simulink model "turbo_controller"  (R2025a)
settings: Solver=FixedStepAuto  StartTime=0.0  StopTime=inf  FixedStep=0.001  RelTol=1e-3
PostLoadFcn:
  | % 自动定位同目录CubeMX文件；不需要外部初始化脚本。
  | codertarget.data.setParameterValue('turbo_controller','STM32CubeMX.ProjectFile',fullfile(fileparts(get_param('turbo_controller','FileName')),'turbo_f407.ioc'));
InitFcn:
  | % 中文说明：按原控制器字段与类型创建三组接口总线；控制参数已内嵌。
  | tc_names=["EValve_Cycle" "EValve_Open" "Eblast_Cycle" "Eblast_Open" "Motor_Cycle" "Motor_Open" "EValve_Enable" "Eblast_Enable" "Motor_Enable" "SWO_Firework" "SWO_BleedAir" "EngineState" "Flag_ECUReset_Clear" "Flag_ECUReset_Save" "Flag_Reset_Enable" "Accelerator" "Nc_dem" "Nc"]; tc_types=["uint16" "uint16" "uint16" "uint16" "uint16" "uint16" "uint8" "uint8" "uint8" "uint8" "uint8" "uint8" "uint8" "uint8" "uint8" "single" "single" "single"];
  | for tc_k=1:numel(tc_names)
  |  tc_e(tc_k)=Simulink.BusElement; tc_e(tc_k).Name=char(tc_names(tc_k)); tc_e(tc_k).DataType=char(tc_types(tc_k));
  | end
  | EngineControl_Out=Simulink.Bus; EngineControl_Out.DataScope='Exported'; EngineControl_Out.Elements=tc_e;
  | clear tc_e tc_names tc_types tc_k
  | tc_names=["savedata1" "savedata2" "savedata3" "savedata4" "savedata5" "savedata6" "savedata7" "savedata8" "savedata9" "savedata10" "savedata11" "savedata12" "savedata13" "savedata14" "savedata15" "savedata16" "savedata17" "savedata18" "savedata19" "savedata20" "savedata21" "savedata22" "savedata23" "savedata24" "savedata25"]; tc_types=["single" "single" "single" "single" "single" "single" "single" "single" "single" "single" "single" "single" "single" "single" "single" "single" "single" "single" "single" "single" "single" "single" "single" "single" "single"];
  | for tc_k=1:numel(tc_names)
  |  tc_e(tc_k)=Simulink.BusElement; tc_e(tc_k).Name=char(tc_names(tc_k)); tc_e(tc_k).DataType=char(tc_types(tc_k));
  | end
  | SaveData_Out=Simulink.Bus; SaveData_Out.DataScope='Exported'; SaveData_Out.Elements=tc_e;
  | clear tc_e tc_names tc_types tc_k
  | tc_names=["senddata1" "senddata2" "senddata3" "senddata4" "senddata5" "senddata6" "senddata7" "senddata8" "senddata9" "senddata10" "senddata11" "senddata12" "senddata13" "senddata14" "senddata15" "senddata16" "senddata17" "senddata18" "senddata19" "senddata20" "senddata21" "senddata22" "senddata23" "senddata24" "senddata25" "senddata26" "senddata27" "senddata28" "senddata29"]; tc_types=["uint8" "uint8" "uint8" "uint8" "uint8" "uint8" "uint8" "uint8" "uint8" "uint8" "uint8" "uint8" "uint8" "uint8" "uint8" "uint8" "uint8" "uint8" "uint8" "uint8" "uint8" "uint8" "uint8" "uint8" "uint8" "uint8" "uint8" "uint8" "uint8"];
  | for tc_k=1:numel(tc_names)
  |  tc_e(tc_k)=Simulink.BusElement; tc_e(tc_k).Name=char(tc_names(tc_k)); tc_e(tc_k).DataType=char(tc_types(tc_k));
  | end
  | SendData_Out=Simulink.Bus; SendData_Out.DataScope='Exported'; SendData_Out.Elements=tc_e;
  | clear tc_e tc_names tc_types tc_k
  | 
  | % 以下为接口中文说明；只设置描述，不改变数值或数据类型。
  | EngineControl_Out.Description='执行控制输出（阀、电机、点火、状态及复位请求）';
  | tc_cn=["EValve_Cycle（主油阀周期计数（每计数2毫秒））" "EValve_Open（主油阀开通计数（每计数2毫秒））" "Eblast_Cycle（副油阀周期计数（每计数2毫秒））" "Eblast_Open（副油阀开通计数（每计数2毫秒））" "Motor_Cycle（起动电机周期计数）" "Motor_Open（起动电机开通计数）" "EValve_Enable（主油阀驱动使能）" "Eblast_Enable（副油阀驱动使能）" "Motor_Enable（起动电机使能）" "SWO_Firework（点火器使能（1开））" "SWO_BleedAir（引气阀使能（1开））" "EngineState（发动机状态）" "Flag_ECUReset_Clear（清除复位恢复状态请求）" "Flag_ECUReset_Save（保存复位恢复数据请求）" "Flag_Reset_Enable（处理器软件复位请求）" "Accelerator（油门／油泵给定控制量）" "Nc_dem（控制目标转速）" "Nc（发动机反馈转速（转每分））"];
  | tc_elements=EngineControl_Out.Elements;
  | for tc_k=1:numel(tc_cn)
  |  tc_elements(tc_k).Description=char(tc_cn(tc_k));
  | end
  | EngineControl_Out.Elements=tc_elements;
  | clear tc_cn tc_elements tc_k
  | SaveData_Out.Description='25项运行记录；字段含义按当前模型数据来源解释';
  | tc_cn=["savedata1（指令回显记录）" "savedata2（入口总温记录（℃））" "savedata3（电源电压记录）" "savedata4（排气温度记录（℃））" "savedata5（标定燃油压力记录）" "savedata6（副油阀占空比记录（％））" "savedata7（主油阀占空比记录（％））" "savedata8（温度修正转速记录）" "savedata9（开关输出及反馈位域）" "savedata10（物理转速记录）" "savedata11（油泵目标给定原始值）" "savedata12（起动电机占空比记录（％））" "savedata13（发动机状态码记录）" "savedata14（故障告警位域记录）" "savedata15（模型记录帧序号）" "savedata16（处理器温度记录（℃））" "savedata17（装订转速记录（沿用旧电源字段名））" "savedata18（导航高度记录）" "savedata19（飞行空速记录）" "savedata20（主阀旧记录位（恒零保留））" "savedata21（第21项保留记录（恒零））" "savedata22（保留记录项22）" "savedata23（保留记录项23）" "savedata24（保留记录项24）" "savedata25（保留记录项25）"];
  | tc_elements=SaveData_Out.Elements;
  | for tc_k=1:numel(tc_cn)
  |  tc_elements(tc_k).Description=char(tc_cn(tc_k));
  | end
  | SaveData_Out.Elements=tc_elements;
  | clear tc_cn tc_elements tc_k
  | SendData_Out.Description='29字段回传及外设命令接口；板端上位机帧只取第3至27字段';
  | tc_cn=["senddata1（回传发送允许标志（不直接上线路））" "senddata2（回传载荷长度25字节）" "senddata3（回传指令回显字节）" "senddata4（总温编码字节（℃＋80））" "senddata5（电源电压编码字节）" "senddata6（排温编码高字节）" "senddata7（排温编码低字节）" "senddata8（燃油压力编码高字节）" "senddata9（燃油压力编码低字节）" "senddata10（副油阀占空比字节（％））" "senddata11（主油阀占空比字节（％））" "senddata12（修正转速编码高字节）" "senddata13（修正转速编码低字节）" "senddata14（驱动及反馈状态位域）" "senddata15（物理转速编码高字节）" "senddata16（物理转速编码低字节）" "senddata17（油泵目标给定高字节（串口二使用））" "senddata18（油泵目标给定低字节（串口二使用））" "senddata19（起动电机占空比命令（串口一使用））" "senddata20（发动机状态码字节）" "senddata21（故障告警位域字节）" "senddata22（帧序号占位（板端另行填写））" "senddata23（处理器温度编码（℃＋50））" "senddata24（控制目标转速编码高字节）" "senddata25（控制目标转速编码低字节）" "senddata26（占位字节（板端改填实测泵速高字节））" "senddata27（占位字节（板端改填实测泵速低字节））" "senddata28（装订转速高字节（本板未发送））" "senddata29（装订转速低字节（本板未发送））"];
  | tc_elements=SendData_Out.Elements;
  | for tc_k=1:numel(tc_cn)
  |  tc_elements(tc_k).Description=char(tc_cn(tc_k));
  | end
  | SendData_Out.Elements=tc_elements;
  | clear tc_cn tc_elements tc_k
  | 
  | 
  | % FRAM模块化事务：接口类型和上电初始状态，随模型保存，无外部初始化文件。
  | clear FM_elements
  | FM_elements(1)=Simulink.BusElement;FM_elements(1).Name='phase';FM_elements(1).DataType='uint8';FM_elements(1).Dimensions=[1 1];FM_elements(1).Description='phase（当前事务阶段）';
  | FM_elements(2)=Simulink.BusElement;FM_elements(2).Name='a';FM_elements(2).DataType='uint8';FM_elements(2).Dimensions=[64 1];FM_elements(2).Description='a（启动时缓存的首区64字节）';
  | FM_elements(3)=Simulink.BusElement;FM_elements(3).Name='active';FM_elements(3).DataType='uint16';FM_elements(3).Dimensions=[1 1];FM_elements(3).Description='active（当前有效记录区地址）';
  | FM_elements(4)=Simulink.BusElement;FM_elements(4).Name='generation';FM_elements(4).DataType='uint32';FM_elements(4).Dimensions=[1 1];FM_elements(4).Description='generation（当前有效记录代号）';
  | FM_elements(5)=Simulink.BusElement;FM_elements(5).Name='record';FM_elements(5).DataType='uint8';FM_elements(5).Dimensions=[64 1];FM_elements(5).Description='record（本次冻结的待写记录）';
  | FM_elements(6)=Simulink.BusElement;FM_elements(6).Name='addr';FM_elements(6).DataType='uint16';FM_elements(6).Dimensions=[1 1];FM_elements(6).Description='addr（本次备用写入地址）';
  | FM_elements(7)=Simulink.BusElement;FM_elements(7).Name='lastSave';FM_elements(7).DataType='single';FM_elements(7).Dimensions=[1 1];FM_elements(7).Description='lastSave（上次开始保存的秒数）';
  | FM_elements(8)=Simulink.BusElement;FM_elements(8).Name='lastState';FM_elements(8).DataType='uint8';FM_elements(8).Dimensions=[1 1];FM_elements(8).Description='lastState（上次保存时的发动机状态）';
  | FM_elements(9)=Simulink.BusElement;FM_elements(9).Name='boot';FM_elements(9).DataType='boolean';FM_elements(9).Dimensions=[1 1];FM_elements(9).Description='boot（启动记录是否允许恢复）';
  | FM_elements(10)=Simulink.BusElement;FM_elements(10).Name='consumed';FM_elements(10).DataType='boolean';FM_elements(10).Dimensions=[1 1];FM_elements(10).Description='consumed（本次启动恢复通知是否已发送）';
  | FM_elements(11)=Simulink.BusElement;FM_elements(11).Name='payload';FM_elements(11).DataType='uint8';FM_elements(11).Dimensions=[20 1];FM_elements(11).Description='payload（当前20字节恢复内容）';
  | ... (+35 lines)
model workspace (MAT data in the model file):
  CRC16_Table_Reference = [0 4129 8258 12387 16516 20645 24774 28903 33032 37161 41290 45419 ... (256 elements, 256x1)]
  PE_Kaer = [0.15402 0.15402 0.12264 0.10076 0.09481 0.07601 0.07111 0.0569 0.05198 0.04926 0.05308 0.04325 ... (13 elements, 1x13)]
  PE_Nr = [21.2982 61.4260372 67.7475458 72.7394382 76.845934 80.6988798 83.8449282 86.6491912 88.9382406 89.178606 91.1938214 93.4068058 ... (13 elements, 1x13)]
  PE_Pump_Translate = 33.5999984741
  PE_RotaSpeed_Translate = 860
  PE_Taer = [0.4939154 0.4939154 0.40780982 0.34066978 0.31622756 0.30405716 0.34300244 0.26785022 0.37393554 0.23914836 0.44563948 0.31044662 ... (13 elements, 1x13)]
  PF_ACCFULLRANGE = 3360
  PF_Flag_ECUReset = 0
  PF_Flag_rx_suc = 1
  PF_Gear_Info = [40000; 45000; 50000; 55000; 57000; 59000; 60000; 61000; 61000; 61000; 61000; 61000]
  PF_K_TiaoJie = 1
  PF_Kpu = 10
  PF_MySet_Rxdata = [0 0 0 0 0 0 0 0 0 0 0 0 ... (50 elements, 50x1)]
  PF_MyUsart1_Rxdata = [0 0 0 0 0 0 0 0 0 0 0 0 ... (50 elements, 50x1)]
  PF_MyUsart2_Rxdata = [0 0 0 0 0 0 0 0 0 0 0 0 ... (50 elements, 50x1)]
  PF_Reset_Information = [0 0 0 0 0 0 0 0 0 0 0 0 ... (20 elements, 20x1)]
  PF_Sensor_X1_T4 = [0 4095]
  PF_Sensor_X2_T4 = [0 1.66666698456]
  PF_Sensor_X3_T4 = [0 504 999 1497 2010 2529 3051 3568 4076 4571 4959]
  PF_Sensor_X_P2 = [0.5 3]
  PF_Sensor_X_Poil = [0.5 3]
  PF_Sensor_X_T1t = [-50 300]
  PF_Sensor_X_Vpower = [0 3]
  PF_Sensor_X_Vpump = [0 3]
  PF_Sensor_Y1_T4 = [0 3]
  PF_Sensor_Y2_T4 = [0 5000]
  PF_Sensor_Y3_T4 = [0 100 200 300 400 500 600 700 800 900 980]
  PF_Sensor_Y_P2 = [0 1000]
  PF_Sensor_Y_Poil = [0 1000]
  PF_Sensor_Y_T1t = [-50 300]
  PF_Sensor_Y_Vpower = [0 33]
  PF_Sensor_Y_Vpump = [0 33]
  PG_CtrlMode_CloseLoop : mpt.Parameter (value not decoded)
  PG_CtrlMode_ManualAcc : mpt.Parameter (value not decoded)
  PG_CtrlMode_Origin : mpt.Parameter (value not decoded)
  PG_CtrlMode_Start : mpt.Parameter (value not decoded)
  PG_CtrlMode_Stop : mpt.Parameter (value not decoded)
  PG_ES_Clp : mpt.Parameter (value not decoded)
  PG_ES_EngStart : mpt.Parameter (value not decoded)
  PG_ES_Manual : mpt.Parameter (value not decoded)
  PG_ES_Origin : mpt.Parameter (value not decoded)
  PG_ES_Stop : mpt.Parameter (value not decoded)
  PG_Instr_BleedAirSet : mpt.Parameter (value not decoded)
  PG_Instr_CloseLoop : mpt.Parameter (value not decoded)
  PG_Instr_ECUReSet : mpt.Parameter (value not decoded)
  PG_Instr_EValveSet : mpt.Parameter (value not decoded)
  PG_Instr_EblastSet : mpt.Parameter (value not decoded)
  PG_Instr_Erase : mpt.Parameter (value not decoded)
  PG_Instr_FireWorkSet : mpt.Parameter (value not decoded)
  PG_Instr_ManualPlus : mpt.Parameter (value not decoded)
  PG_Instr_ManualrReduce : mpt.Parameter (value not decoded)
  PG_Instr_MotorSet : mpt.Parameter (value not decoded)
  PG_Instr_OilSet : mpt.Parameter (value not decoded)
  PG_Instr_SelfCheck : mpt.Parameter (value not decoded)
  PG_Instr_Start : mpt.Parameter (value not decoded)
  PG_Instr_Stop : mpt.Parameter (value not decoded)
  PG_Instr_StopZero : Simulink.Parameter (value not decoded)
  PG_Location_Air : Simulink.Parameter (value not decoded)
  PG_Location_Gnd : Simulink.Parameter (value not decoded)
  PG_ServoCtrlMode_CloseLoop : Simulink.Parameter (value not decoded)
  PG_ServoCtrlMode_CloseLoopMax : Simulink.Parameter (value not decoded)
  PG_ServoCtrlMode_CloseLoopMin : Simulink.Parameter (value not decoded)
  PG_ServoCtrlMode_ManualAcc : Simulink.Parameter (value not decoded)
  PG_ServoCtrlMode_ManualAccMax : Simulink.Parameter (value not decoded)
  PG_ServoCtrlMode_ManualAccMin : Simulink.Parameter (value not decoded)
  PG_SpeedDot_Permit : Simulink.Parameter (value not decoded)
  PL_EngineModel_Actuator = [0 10 100]
  PL_EngineModel_EngineStar_Press_P2 = [1013 1098.4 1099.144828 1099.931034 1103.613793 1162.662069 1143.793103 1131.006897 1123.186207 1117.6 1114 1111.806897 ... (127 elements, 1x127)]
  PL_EngineModel_EngineStar_RotaSpeed = [200 2000 9584 9660 10220 10240 10260 10288 10308 10368 10380 10408 ... (127 elements, 1x127)]
  PL_EngineModel_EngineStar_Temp_Exhaust = [128 129 129.1 130 131 131.1 132 133 134 134.1 135 135.1 ... (127 elements, 1x127)]
  PL_EngineModel_EngineStar_Time = [0.05 0.1 0.15 0.2 0.25 0.3 0.35 0.4 0.45 0.5 0.55 0.6 ... (127 elements, 1x127)]
  PL_EngineModel_IdleAbove_Nr = [0 21.2982 61.4260372 67.7475458 72.7394382 76.845934 80.6988798 83.8449282 86.6491912 88.9382406 89.178606 91.1938214 ... (14 elements, 1x14)]
  PL_EngineModel_IdleAbove_P2r = [0.986923266716 1.57907722675 1.81593881076 1.99358499877 2.23044658278 2.43770046879 2.65482358747 2.84233900814 3.03972366149 3.18776215149 3.25684678016 3.3950160375 ... (14 elements, 1x14)]
  PL_EngineModel_IdleAbove_Tempr = [0.0536001429337 1.07200285867 1.63301768805 1.63659103091 1.66875111667 1.72592460247 1.77595140254 1.86171163123 1.95461854565 2.03323208862 2.03323208862 2.13685903162 ... (14 elements, 1x14)]
  PL_EngineModel_IdleAbove_Ter = [0.42434128 0.42434128 0.42434128 0.30669408 0.23570008 0.22150128 0.1997974 0.23803274 0.16115638 0.24279948 0.13600422 0.31308354 ... (14 elements, 1x14)]
  PL_EngineModel_IdleAbove_Wfr = [0 10.142 23.8337 27.8905 31.9473 36.0041 40.0609 44.1177 48.1745 52.2313 52.7384 56.7952 ... (14 elements, 1x14)]
  PL_EngineModel_Press_P2 = [400 400 400 400 400 400 400 400 400 400]
  PL_EngineModel_Rotaspeed = [0 20000 96400]
  PL_EngineModel_Temp_Exhaust = [500 500 500 500 500 500 500 500 500 500]
  PL_Kaer = [0.1 0.1 0.1 0.1 0.1 0.1]
  PL_Nr = [50 60 70 80 90 100]
  PL_Taer = [0.1 0.1 0.1 0.1 0.1 0.1]
  Sig : Simulink.Signal (value not decoded)
  Ts_ms : Simulink.Parameter (value not decoded)
  false : Simulink.Parameter (value not decoded)
  true : Simulink.Parameter (value not decoded)
symbols that are objects in the model workspace (value not decoded): PG_CtrlMode_CloseLoop, PG_CtrlMode_ManualAcc, PG_CtrlMode_Origin, PG_CtrlMode_Start, PG_CtrlMode_Stop, PG_ES_Clp, PG_ES_EngStart, PG_ES_Manual, PG_ES_Origin, PG_ES_Stop, PG_Instr_BleedAirSet, PG_Instr_CloseLoop, PG_Instr_EblastSet, PG_Instr_ECUReSet, PG_Instr_Erase, PG_Instr_EValveSet, PG_Instr_FireWorkSet, PG_Instr_ManualPlus, PG_Instr_ManualrReduce, PG_Instr_MotorSet, PG_Instr_OilSet, PG_Instr_SelfCheck, PG_Instr_Start, PG_Instr_Stop, PG_Instr_StopZero, PG_ServoCtrlMode_CloseLoop, PG_ServoCtrlMode_CloseLoopMax, PG_ServoCtrlMode_CloseLoopMin, PG_ServoCtrlMode_ManualAcc, PG_ServoCtrlMode_ManualAccMax, PG_ServoCtrlMode_ManualAccMin, Ts_ms
libraries: simulink x97, stm32blockslib x10, stm32f4xxblockslib x8
(part 10 of 26)

== system turbo_controller/ESM/Flags ==
  note: 把分散的进入条件整理为11个模式转换标志
      |
      | 分别检查初始到起动、初始到手动、进入闭环、各模式停车、停车回初始等条件，再将11个布尔结果打
      | 成Flags总线交状态机使用。
      |
      | 例如普通起动要求Start命令且转速不超过13000；停车回初始要求停车完成且转速不超过20000。部分
      | 控制分支结果先经过一拍延迟再反馈，防止同一拍组合判断互相循环。
      |
      | 这里的每一项是“是否允许这条转换”，不是发动机模式本身，也不是报警编号。真正的当前模式由St
      | ateTranslation保存。
  S_Nc : Inport
      settings: AttributesFormatString=S_Nc（发动机反馈转速（转每分））
  S_Instr : Inport  Port=2
      settings: AttributesFormatString=S_Instr（指令）
  S_Flag_ECUReset : Inport  Port=3
      settings: AttributesFormatString=S_Flag_ECUReset（复位恢复标志）
  S_CLM_Parameter : Inport  Port=4
      settings: AttributesFormatString=S_CLM_Parameter（控制规律管理模块参数）
  Bus Creator1 : BusCreator  Inputs=11
      settings: AttributesFormatString=Bus Creator1（总线创建器1）
  Bus Selector2 : BusSelector  OutputSignals=S_Start（地面起动参数总线）.Flag_RunState（运行状态标志）,S_Stop（停车参数总线）.StopFinish（停车完成标志）
      settings: AttributesFormatString=Bus Selector2（总线选择器2）
  EngineClp : Subsystem  Description=|
      | 产生进入闭环模式的允许条件
      | 
      | 起动分支的阶段结果达到2时，产生Start到Clp条件；手动到Clp使用闭环命令判断；初始到Clp保留复位恢复有效条件。
      | 
      | 同一个“进入闭环”请求，在不同来源模式下有不同条件，不能只看当前目标转速非零就进入闭环。本处只输出转换许可，StateTranslation还要结合当前状态决定采用哪条转换。当前恢复标志上层未启用，恢复进入闭环路径不会自动投入。
      settings: AttributesFormatString=EngineClp（闭环状态转换判定）
  EngineOrigin : Subsystem  Description=|
      | 判断停车结束后是否可以回到初始模式
      | 
      | 只有StopFinish为真，且当前转速Nc≤20000 rpm，两项同时满足才输出Stop2Origin。停车图完成但转速仍很高时，不立即给出这个许可。
      | 
      | 这里不主动制动，也不强迫传感器转速归零。“回初始”是控制流程退出停车模式，不等同于轴已经完全静止。StateTranslation在当前确实处于Stop时才会使用这条转换条件。
      settings: AttributesFormatString=EngineOrigin（原位状态转换判定）
  EngineStart : Subsystem  Description=|
      | 判断能否开始普通起动
      | 
      | 命令必须等于PG_Instr_Start，同时当前转速Nc≤13000 rpm。两项同时成立才输出Origin2Start；其他命令或转速过高时不允许这条转换。
      | 
      | 这只是从初始模式进入普通起动的门槛。点火、建压、供油和退出电机由Start内部顺序图接着执行，不能把13000理解为起动完成转速。工程当前只保留普通Start，不含空气或丙烷起动分支。
      settings: AttributesFormatString=EngineStart（起动状态转换判定）
  EngineStop : Subsystem  Description=|
      | 把停车命令和起动异常转换成停车请求
      | 
      | Stop和StopZero命令都可形成相应停车转换条件；起动内部阶段结果4或15也参与起动转停车判断，用于流程异常或退出。
      | 
      | 分别输出Clp2Stop、Manual2Stop、Start2Stop，交状态机按当前模式选择。内部阶段结果15并不是对外EngineState=15；对外停车模式编号仍为4。
      | 
      | 本模块只提出转换要求，停车后关闭油路、是否短时拖转及何时完成由Stop分支处理。
      settings: AttributesFormatString=EngineStop（停车状态转换判定）
  Manual : Subsystem  Description=|
      | 识别会进入手动模式的八类命令
      | 
      | 比较当前命令是否属于手动泵直接设定、加、减、主油阀、副油阀、起动电机、点火器或引气阀设置。任一匹配便形成进入手动的条件。
      | 
      | 分别向初始、起动、闭环模式提供转Manual标志，真正能用哪一条由状态机的当前状态决定。这里不解释Data6的开度和数值；进入手动后，CLM/Manual才把命令参数换成具体执行器设定。
      settings: AttributesFormatString=Manual（手动）
  Time Delay1 : UnitDelay  SampleTime=-1  HasFrameUpgradeWarning=on
      settings: AttributesFormatString=Time Delay1（时间延迟1）
  Time Delay2 : UnitDelay  SampleTime=-1  HasFrameUpgradeWarning=on
      settings: AttributesFormatString=Time Delay2（时间延迟2）
  Time Delay8 : UnitDelay  SampleTime=-1  HasFrameUpgradeWarning=on
      settings: AttributesFormatString=Time Delay8（时间延迟8）
  S_Flags : Outport
      settings: AttributesFormatString=S_Flags（标志集合）
  wires:
  S_Instr/1 -> EngineStop/2(S_Instr), EngineClp/2(S_Instr), EngineStart/1(S_Instr), Manual/1(S_Instr)
  EngineStart/1(S_Origin2Start) -> [Origin2Start]
  EngineStop/1(S_Clp2Stop) -> [Clp2Stop]
  Manual/1(S_Start2Manual) -> [Start2Manual]
  Manual/2(S_Clp2Manual) -> [Clp2Manual]
  EngineStop/2(S_Manual2Stop) -> [Manual2Stop]
  EngineClp/2(S_Manual2Clp) -> [Manual2Clp]
  S_Flag_ECUReset/1 -> EngineClp/3(S_Flag_ECUReset)
  EngineClp/3(S_Origin2Clp) -> [Origin2Clp]
  EngineStop/3(S_Start2Stop) -> [Start2Stop]
  Manual/3(S_Origin2Manual) -> [Origin2Manual]
  S_CLM_Parameter/1 -> Bus Selector2/1
  Bus Selector2/1 -> Time Delay8/1, Time Delay2/1  "<Flag_RunState（运行状态标志）>"
  Time Delay8/1 -> EngineStop/1(S_Flag_EnigneState)
  EngineClp/1(S_Start2Clp) -> [Start2Clp]
  Time Delay2/1 -> EngineClp/1(S_Flag_EnigneState)
  [Origin2Manual] -> Bus Creator1/11  "Origin2Manual（原位转手动条件）"
  [Origin2Clp] -> Bus Creator1/10  "Origin2Clp（原位转闭环条件）"
  [Start2Stop] -> Bus Creator1/9  "Start2Stop（地面起动转停车条件）"
  [Clp2Manual] -> Bus Creator1/8  "Clp2Manual（闭环转手动条件）"
  [Start2Manual] -> Bus Creator1/7  "Start2Manual（地面起动转手动条件）"
  [Manual2Stop] -> Bus Creator1/6  "Manual2Stop（手动转停车条件）"
  [Manual2Clp] -> Bus Creator1/5  "Manual2Clp（手动转闭环条件）"
  [Stop2Origin] -> Bus Creator1/4  "Stop2Origin（停车转原位条件）"
  [Clp2Stop] -> Bus Creator1/3  "Clp2Stop（闭环转停车条件）"
  [Start2Clp] -> Bus Creator1/2  "Start2Clp（地面起动转闭环条件）"
  [Origin2Start] -> Bus Creator1/1  "Origin2Start（原位转地面起动条件）"
  Bus Selector2/2 -> Time Delay1/1  "<StopFinish（停车完成标志）>"
  Time Delay1/1 -> EngineOrigin/2(S_StopFinish)
  EngineOrigin/1(S_Stop2Origin) -> [Stop2Origin]
  S_Nc/1 -> EngineOrigin/1(S_Nc), EngineStart/2(S_Nc)
  Bus Creator1/1 -> S_Flags/1

== system turbo_controller/ESM/StateTransition ==
  note: 管理发动机运行模式，而不是直接控制驱动电平
      |
      | Flags先根据命令、当前转速、起动阶段结果、停车完成标志及恢复条件，计算允许发生哪些模式转换
      | 。StateTranslation再按当前所在模式和这些允许条件切换状态。
      |
      | 对外只有五种运行模式：Origin=0、Start=1、Clp=2、Manual=3、Stop=4。普通起动内部的A～F及异常
      | 阶段码不属于这五个模式编号。
      |
      | 输出EngineState供CLM选择相应控制分支，供通信与记录解释运行状态。本层不生成泵字节或GPIO脉冲
      | ；转换进入Start仅表示开始执行起动分支，不代表已达到闭环转速。
  S_Flags : Inport
      settings: AttributesFormatString=S_Flags（标志集合）
  Bus Selector1 : BusSelector  OutputSignals=Origin2Start（原位转地面起动条件）,Start2Clp（地面起动转闭环条件）,Clp2Stop（闭环转停车条件）,Stop2Origin（停车转原位条件）,Manual2Clp（手动转闭环条件）,Manual2Stop（手动转停车条件）,Start2Manual（地面起动转手动条件）,Clp2Manual（闭环转手动条件）,Start2Stop（地面起动转停车条件）,Origin2Clp（原位转闭环条件）,Origin2Manual（原位转手动条件）
      settings: AttributesFormatString=Bus Selector1（总线选择器1）
  StateTranslation : Stateflow chart  Description=|  TreatAsAtomicUnit=on
      | 保存五种发动机模式，并按允许条件切换
      | 
      | 初始为Origin，对外编号0。收到相应转换标志后，可以进入普通Start=1、闭环Clp=2或手动Manual=3；运行过程中停车请求进入Stop=4，停车完成并满足转速条件再回Origin。
      | 
      | 每个状态的进入动作写EngineState，其他子系统读取这个编号决定运行哪套控制算法。转换的守卫条件来自Flags，起动是否完成则来自Start内部阶段结果。
      | 
      | 本图是模式记忆：即便某个命令只出现一拍，已进入的模式也会保持到下一次合法转换。不能把命令编号、起动A～F阶段和这五种模式当作同一种“状态”。
      settings: AttributesFormatString=StateTranslation（状态转换）
  S_EngineState : Outport
      settings: AttributesFormatString=S_EngineState（发动机状态）
  wires:
  Bus Selector1/11 -> StateTranslation/11(Origin2Manual)  "<Origin2Manual（原位转手动条件）>"
  Bus Selector1/10 -> StateTranslation/10(Origin2Clp)  "<Origin2Clp（原位转闭环条件）>"
  Bus Selector1/9 -> StateTranslation/9(Start2Stop)  "<Start2Stop（地面起动转停车条件）>"
  Bus Selector1/8 -> StateTranslation/8(Clp2Manual)  "<Clp2Manual（闭环转手动条件）>"
  Bus Selector1/7 -> StateTranslation/7(Start2Manual)  "<Start2Manual（地面起动转手动条件）>"
  Bus Selector1/6 -> StateTranslation/6(Manual2Stop)  "<Manual2Stop（手动转停车条件）>"
  Bus Selector1/5 -> StateTranslation/5(Manual2Clp)  "<Manual2Clp（手动转闭环条件）>"
  StateTranslation/1(EngineState) -> S_EngineState/1
  Bus Selector1/4 -> StateTranslation/4(Stop2Origin)  "<Stop2Origin（停车转原位条件）>"
  Bus Selector1/3 -> StateTranslation/3(Clp2Stop)  "<Clp2Stop（闭环转停车条件）>"
  Bus Selector1/2 -> StateTranslation/2(Start2Clp)  "<Start2Clp（地面起动转闭环条件）>"
  Bus Selector1/1 -> StateTranslation/1(Origin2Start)  "<Origin2Start（原位转地面起动条件）>"
  S_Flags/1 -> Bus Selector1/1

== system turbo_controller/FPM/Subsystem ==
  note: 极值斜率故障
  note: 故障锁存标志
  note: ACDC转速启动前可能乱跳，造成故障锁定
  note: 【本页库子系统中文说明】Detect
      | Change
      | 一、它做什么？
      | 比较当前输入与上一次输入是否不同：发生变化时给出变化标志，不变时不给出变化标
      | 志。它检测的是数值改变，不是判断数值够不够大。内部需要记住上次输入，首次输出
      | 还要结合库块的初值设置。
      | 二、本实例当前参数
      | vinit：0
      | InputProcessing：Elements as channels (sample based)
      | 输出数据类型：布尔值，真或假
      | 三、怎样继续学习？
      | 这是标准库子系统实例。中文说明放在使用它的父级页面，并同步存入本块Descriptio
      | n（模块说明）；官方库链接保留。先看本实例的输入来自哪里、输出交给谁，再结合
      | 以上参数理解作用。
  note: 【本页库子系统中文说明】运行状态
      | 一、它做什么？
      | 这是“过不过这条线”的判断器。将输入与阈值 PG_ES_Clp 作 == 比较，关系成立输
      | 出真（1），否则输出假（0）。例如>=包含恰好等于，>则不包含。它只给出判断标志
      | ，不会自行限幅、报警、切换状态或操作阀门；后续逻辑决定如何使用。名称可能只是
      | 用途提示，实际判据以这里的关系和阈值为准。
      | 二、本实例当前参数
      | 比较关系：==
      | 比较阈值：PG_ES_Clp
      | 输出数据类型：uint8
      | 零交叉检测：开启
      | 三、怎样继续学习？
      | 这是标准库子系统实例。中文说明放在使用它的父级页面，并同步存入本块Descriptio
      | n（模块说明）；官方库链接保留。先看本实例的输入来自哪里、输出交给谁，再结合
      | 以上参数理解作用。
  note: 【本页库子系统中文说明】闭环状态
      | 一、它做什么？
      | 这是“过不过这条线”的判断器。将输入与阈值 PG_ES_Clp 作 == 比较，关系成立输
      | 出真（1），否则输出假（0）。例如>=包含恰好等于，>则不包含。它只给出判断标志
      | ，不会自行限幅、报警、切换状态或操作阀门；后续逻辑决定如何使用。名称可能只是
      | 用途提示，实际判据以这里的关系和阈值为准。
      | 二、本实例当前参数
      | 比较关系：==
      | 比较阈值：PG_ES_Clp
      | 输出数据类型：uint8
      | 零交叉检测：开启
      | 三、怎样继续学习？
      | 这是标准库子系统实例。中文说明放在使用它的父级页面，并同步存入本块Descriptio
      | n（模块说明）；官方库链接保留。先看本实例的输入来自哪里、输出交给谁，再结合
      | 以上参数理解作用。
  note: 区分短时测速异常、持续故障和恢复保存时机
      |
      | 把转速幅值故障与突变故障组合，先形成当前异常，再经10 s定时锁存形成持续故障。暂时异常可让控
      | 制保持，持续异常则允许父级切换备份供油策略。
      |
      | 恢复有效条件持续约2 s后产生恢复工作相关状态；处于闭环时，4 s计时器周期性给出保存事件。模式
      | 变化检测与触发/使能分支产生恢复信息清除请求。
      |
      | 这些都是控制条件，不是FRAM写入已完成的确认。实际保存需要下游事务逐步执行，写失败也不能仅靠
      | 本模块得知。
  note: Detect
      | Change
      | 检测发动机模式是否与上一拍不同
      |
      | 输入为当前模式，与内部保存的上次值比较，变化时输出真，未变化时输出假。初始比较值为0，所以
      | 首次输入0不算变化，首次输入非0会触发。
      |
      | 这是变化事件，不是持续处于某模式的标志。父级用它安排复位恢复信息清除等动作；本实例不直接清
      | 除FRAM，也不会持续一整个模式都重复触发。
  note: 运行状态
      | 运行状态：只判断一个条件
      |
      | 把输入与2比较，使用关系“==”。成立输出1，不成立输出0；输出是判断标志，不是把输入缩放成该
      | 常数。
      |
      | 这里比较的是发动机当前模式：初始0、普通起动1、闭环2、手动3、停车4。结果供父级选择对应控制/
      | 保护路径，不能用命令编号代替模式编号。
  note: 闭环状态
      | 闭环状态：只判断一个条件
      |
      | 把输入与2比较，使用关系“==”。成立输出1，不成立输出0；输出是判断标志，不是把输入缩放成该
      | 常数。
      |
      | 这里比较的是发动机当前模式：初始0、普通起动1、闭环2、手动3、停车4。结果供父级选择对应控制/
      | 保护路径，不能用命令编号代替模式编号。
  In1 : Inport
      settings: AttributesFormatString=In1（输入1）
  In2 : Inport  Port=2
      settings: AttributesFormatString=In2（输入2）
  Bus Selector1 : BusSelector  OutputSignals=Sensor（传感器信息总线）.Nc_Flag_Locking（转速信号锁定标志）,Sensor（传感器信息总线）.Ncdot_Flag_Locking（转速变化率锁定标志）
      settings: AttributesFormatString=Bus Selector1（总线选择器1）
  Bus Selector2 : BusSelector  OutputSignals=COMM（通信信息总线）.Flag_ECUReset_Use（复位恢复数据使用标志）
      settings: AttributesFormatString=Bus Selector2（总线选择器2）
  Constant4 : Constant  Value=10000  OutDataTypeStr=single  SampleTime=-1
      settings: AttributesFormatString=Constant4（常量4）
  Data Type Conversion{1..5} (5 alike) : DataTypeConversion  OutDataTypeStr=uint8  SaturateOnIntegerOverflow=off  RndMeth=Floor
      Data Type Conversion1 settings: AttributesFormatString=Data Type Conversion1（数据类型转换1）
      Data Type Conversion2 settings: AttributesFormatString=Data Type Conversion2（数据类型转换2）
      Data Type Conversion3 settings: AttributesFormatString=Data Type Conversion3（数据类型转换3）
      Data Type Conversion4 settings: AttributesFormatString=Data Type Conversion4（数据类型转换4）
      Data Type Conversion5 settings: AttributesFormatString=Data Type Conversion5（数据类型转换5）
  Detect Change : simulink/Logic and Bit Operations/Detect Change  Description=|  vinit=0  OutDataTypeStr=boolean
      | 检测发动机模式是否与上一拍不同
      | 
      | 输入为当前模式，与内部保存的上次值比较，变化时输出真，未变化时输出假。初始比较值为0，所以首次输入0不算变化，首次输入非0会触发。
      | 
      | 这是变化事件，不是持续处于某模式的标志。父级用它安排复位恢复信息清除等动作；本实例不直接清除FRAM，也不会持续一整个模式都重复触发。
      settings: AttributesFormatString=Detect Change（检测变化）
  Flag_ECUReset_Reset : Subsystem  Description=|  TreatAsAtomicUnit=on
      | 在被触发且允许时提出恢复记录清除请求
      | 
      | 这是带触发和使能的动作子系统。只有父级满足执行条件时，内部常量1才输出为清除请求；不是模型每拍都无条件清除FRAM。
      | 
      | 本处不发送SPI、不擦除整片存储器，只生成逻辑标志。父级将它与模式变化等条件组合，再由FRAM事务层决定实际记录处理。
      settings: AttributesFormatString=Flag_ECUReset_Reset（标志控制器复位复位）
  Hold_2000ms : Stateflow chart  Description=|  TreatAsAtomicUnit=on  RTWFcnName=Timmer  RTWFileName=MCM_Timmer
      | 等待恢复条件持续约2 s后才置恢复控制标志
      | 
      | Flag_ECUReset为真时累计次数，为假时立即清计数并令ResetControl为假。计数尚小于Time_ms/Ts_ms时输出假，达到门限后输出真。
      | 
      | 当前Time_ms=2000、Ts_ms=20，对应100次调用。这样一次瞬时有效信号不会立即完成恢复确认。计数有10000封顶，避免持续有效时无限增长；输入撤销后需要重新累计。
      settings: AttributesFormatString=Hold_2000ms（保持2000毫秒）  RTWFcnNameOpts=Use subsystem name  RTWFileNameOpts=User specified
  Hold_4000ms : Stateflow chart  Description=|  TreatAsAtomicUnit=on  RTWFcnName=Timmer  RTWFileName=MCM_Timmer
      | 闭环期间按约4 s间隔提出保存请求
      | 
      | Flag_ClpControl为真时计数，为假时清零且不保存。当计数严格大于Time_ms/Ts_ms时，ECUReset_Save给出真并清计数，随后重新开始下一轮。
      | 
      | 当前Time_ms=4000、Ts_ms=20，比较门限200次，因采用“>”，事件会比恰好200拍多一个调用量级。它是周期性的保存触发，不是持续4 s都在发写命令。真正的多步FRAM写入由事务子系统完成。
      settings: AttributesFormatString=Hold_4000ms（保持4000毫秒）  RTWFcnNameOpts=Use subsystem name  RTWFileNameOpts=User specified
  Logical Operator1 : Logic  Operator=OR  AllPortsSameDT=off  OutDataTypeStr=boolean
      settings: AttributesFormatString=Logical Operator1（逻辑运算1）
  Logical Operator2 : Logic  Operator=OR  AllPortsSameDT=off  OutDataTypeStr=boolean
      settings: AttributesFormatString=Logical Operator2（逻辑运算2）
  Logical Operator3 : Logic  Operator=NOT  AllPortsSameDT=off  OutDataTypeStr=boolean
      settings: AttributesFormatString=Logical Operator3（逻辑运算3）
  Logical Operator4 : Logic  AllPortsSameDT=off  OutDataTypeStr=boolean
      settings: AttributesFormatString=Logical Operator4（逻辑运算4）
  Logical Operator5 : Logic  AllPortsSameDT=off  OutDataTypeStr=boolean
      settings: AttributesFormatString=Logical Operator5（逻辑运算5）
  Scope : Scope
      settings: AttributesFormatString=Scope（示波器）  ActiveDisplayYMinimum=-0.125  ActiveDisplayYMaximum=1.125  DataLoggingVariableName=ScopeData4
  Timmer_ms_Lock : Stateflow chart  Description=|  TreatAsAtomicUnit=on  RTWFcnName=Timmer  RTWFileName=EngineControl_Timmer
      | 持续异常达到时间门限后锁存故障
      | 
      | 输入In为真或内部Flag_Lock已经为真时计数。计数严格大于Time_ms/Ts_ms后，置Out和Flag_Lock为真。锁存之后，即便外部In恢复为假，也继续维持故障状态，直到模型/图初始化。
      | 
      | 父级Time_ms=10000、Ts_ms=20，门限500次调用，采用“>”判断。这样短暂测速异常先走临时保护，持续约10 s才进入长期故障策略。计数有上限，不无限累加。
      settings: AttributesFormatString=Timmer_ms_Lock（计时器毫秒锁存）  RTWSystemCode=Reusable function  RTWFcnNameOpts=Use subsystem name  RTWFileNameOpts=User specified
  dth = T0-288.1 : Constant  Value=4000  OutDataTypeStr=single  SampleTime=-1
      settings: AttributesFormatString=dth = T0-288.1（固定常量4000（旧名称不参与计算））
  dth = T0-288.5 : Constant  Value=2000  OutDataTypeStr=single  SampleTime=-1
      settings: AttributesFormatString=dth = T0-288.5（固定常量2000（旧名称不参与计算））
  运行状态 : simulink/Logic and Bit Operations/Compare To Constant  Description=|  relop===  const=PG_ES_Clp  OutDataTypeStr=uint8
      | 运行状态：只判断一个条件
      | 
      | 把输入与2比较，使用关系“==”。成立输出1，不成立输出0；输出是判断标志，不是把输入缩放成该常数。
      | 
      | 这里比较的是发动机当前模式：初始0、普通起动1、闭环2、手动3、停车4。结果供父级选择对应控制/保护路径，不能用命令编号代替模式编号。
  闭环状态 : simulink/Logic and Bit Operations/Compare To Constant  Description=|  relop===  const=PG_ES_Clp  OutDataTypeStr=uint8
      | 闭环状态：只判断一个条件
      | 
      | 把输入与2比较，使用关系“==”。成立输出1，不成立输出0；输出是判断标志，不是把输入缩放成该常数。
      | 
      | 这里比较的是发动机当前模式：初始0、普通起动1、闭环2、手动3、停车4。结果供父级选择对应控制/保护路径，不能用命令编号代替模式编号。
  Lock_NcFailure : Outport
      settings: AttributesFormatString=Lock_NcFailure（锁存转速故障）
  Flag_NcFailure1 : Outport  Port=2
      settings: AttributesFormatString=Flag_NcFailure1（标志转速故障1）
  Flag_ECUReset_work : Outport  Port=3
      settings: AttributesFormatString=Flag_ECUReset_work（标志控制器复位工作）
  Flag_ECUReset_Clear : Outport  Port=4
      settings: AttributesFormatString=Flag_ECUReset_Clear（清除复位恢复状态请求）
  Flag_ECUReset_Save : Outport  Port=5
      settings: AttributesFormatString=Flag_ECUReset_Save（保存复位恢复数据请求）
  wires:
  Logical Operator2/1 -> Logical Operator5/2, Logical Operator4/2, Scope/1
  Bus Selector2/1 -> Flag_ECUReset_Reset/Enable, Hold_2000ms/1(Flag_ECUReset)  "<Flag_ECUReset_Use（复位恢复数据使用标志）>"
  In1/1 -> Bus Selector1/1, Bus Selector2/1
  Bus Selector1/1 -> Logical Operator2/1  "<Nc_Flag_Locking（转速信号锁定标志）>"
  Bus Selector1/2 -> Logical Operator2/2  "<Ncdot_Flag_Locking（转速变化率锁定标志）>"
  Hold_2000ms/1(ResetControl) -> Flag_ECUReset_Reset/Trigger, Data Type Conversion1/1
  Flag_ECUReset_Reset/1(S_Flag_ECUReset_Clear) -> Logical Operator1/1
  dth = T0-288.5/1 -> Hold_2000ms/2(Time_ms)
  Detect Change/1 -> Logical Operator1/2
  闭环状态/1 -> Hold_4000ms/1(Flag_ClpControl)
  Hold_4000ms/1(ECUReset_Save) -> Data Type Conversion5/1  "Flag_ECUReset_Save（保存复位恢复数据请求）"
  Data Type Conversion2/1 -> Flag_ECUReset_Clear/1  "Flag_ECUReset_Clear（清除复位恢复状态请求）"
  Logical Operator1/1 -> Data Type Conversion2/1
  dth = T0-288.1/1 -> Hold_4000ms/2(Time_ms)
  Data Type Conversion1/1 -> Flag_ECUReset_work/1  "Flag_ECUReset_work（复位恢复运行标志）"
  Timmer_ms_Lock/1(Out) -> Logical Operator3/1, Data Type Conversion3/1
  Constant4/1 -> Timmer_ms_Lock/2(Time_ms)
  In2/1 -> 运行状态/1, 闭环状态/1, Detect Change/1
  运行状态/1 -> Logical Operator4/1
  Logical Operator4/1 -> Timmer_ms_Lock/1(In)
  Data Type Conversion4/1 -> Flag_NcFailure1/1
  Data Type Conversion5/1 -> Flag_ECUReset_Save/1
  Data Type Conversion3/1 -> Lock_NcFailure/1
  Logical Operator3/1 -> Logical Operator5/1
  Logical Operator5/1 -> Data Type Conversion4/1

== system turbo_controller/SDM/LogicSelection3 ==
  note: 根据条件选择两种检测结果
      |
      | C不为0时输出T，C为0时输出F。父级用它在不同运行条件下选择相应检测结果；不把两路标志相加，也
      | 不保存上次值。
      |
      | 本处只处理选择，具体检测阈值在T4_Check及父级比较模块中。当前整个SDM结果最终接到未使用终止
      | 端，因此此选择不会单独触发实际停车或起动。
  C : Inport
      settings: AttributesFormatString=C（条件输入或阶段编号）
  F : Inport  Port=2
      settings: AttributesFormatString=F（假分支输入）
  T : Inport  Port=3
      settings: AttributesFormatString=T（温度、时间或真分支输入）
  Switch : Switch  Criteria=u2 ~= 0  SaturateOnIntegerOverflow=off  InputSameDT=off
      settings: AttributesFormatString=Switch（开关选择）
  Out : Outport
      settings: AttributesFormatString=Out（输出）
  wires:
  F/1 -> Switch/3
  T/1 -> Switch/1
  C/1 -> Switch/2
  Switch/1 -> Out/1

== system turbo_controller/SDM/T4_Check ==
  note: 用排温是否超过100判断升温条件
      |
      | 读取排温并与100比较，输出该比较条件供SDM组合使用。这里采用已送入本模块的温度量，不直接读取
      | ADC计数，也不重新执行传感器标定。
      |
      | 阈值判断仅表示温度位于门限哪一侧，没有持续2 s确认，也不是完整的点火成功识别。当前SDM输出未
      | 继续参与模式控制，不能把本标志视为已经投入的起动保护。
  In1 : Inport
      settings: AttributesFormatString=In1（输入1）
  Constant7 : Constant  Value=100
      settings: AttributesFormatString=Constant7（常量7）
  Data Type Conversion4 : DataTypeConversion  OutDataTypeStr=uint8  SaturateOnIntegerOverflow=off  RndMeth=Floor
      settings: AttributesFormatString=Data Type Conversion4（数据类型转换4）
  Relational Operator5 : RelationalOperator  Operator=>  OutDataTypeStr=boolean  InputSameDT=off
      settings: AttributesFormatString=Relational Operator5（关系比较运算5）
  Out1 : Outport
      settings: AttributesFormatString=Out1（输出1）
  wires:
  Constant7/1 -> Relational Operator5/2
  In1/1 -> Relational Operator5/1
  Relational Operator5/1 -> Data Type Conversion4/1
  Data Type Conversion4/1 -> Out1/1

== system turbo_controller/BoardInput_输入换算与协议解析/In01_Host（上位机命令解析）/Receive（逐字节组帧与保持有效结果）_108 ==
  note: 上位机接收流程：按1→2→3→4阅读，第5步管理通知时机
      |
      | 这页只保留三个输入、两个输出、一个循环块和五个处理步骤。
      | Rx：接收数组；Count：本批新收到多少字节；ControlTick：20 ms更新许可。
      | Command：最近有效的50项命令；Flag：本次是否通知控制任务有新命令。
      |
      | Step01取一项字节，决定本项有效及何时结束循环。
      | Step02识别AA55并拼14字节，未拼完的数据保留到下次。
      | Step03检查收齐事件及累加、异或校验，给出本次接受事件。
      | Step04有效才更新命令，否则保持上一条；14字节后补36个0。
      | Step05记住是否有新命令，等20 ms许可时输出通知。
      |
      | 三种记忆各管一件事：半帧缓存属于Step02；上一条有效命令属于Step04；尚未报告标志属于Step05。
      | 候选帧、有效命令、通知标志不能混为一谈。
      |
      | Loop让这五步在本次调用内逐字节重复，不是五步各等一个采样周期。Step01的下一序号反馈Loop，达
      | 到本批数量或64项就结束。因此一批能处理多字节，也能连续接受多帧。
      |
      | 本次仅拆分层次，保留原来的循环、类型转换、初值、校验与保持逻辑。点开每一步可看具体例子及输
      | 入输出含义。
  Rx（本次接收字节）_11 : Inport  OutDataTypeStr=uint8
  Count（本次有效字节数）_12 : Inport  Port=2  OutDataTypeStr=uint32
  ControlTick（20毫秒更新许可）_13 : Inport  Port=3  OutDataTypeStr=boolean
  Loop（逐项处理循环）_14 : ForIterator  IterationLimit=64  ExternalIncrement=on  IterationVariableDataType=uint32
  Step01_取字节与循环控制 : Subsystem  Description=|
      | 第一步：从本批数据中逐个取字节，决定何时结束循环
      | 
      | Rx是最多64项的接收数组，Count说明其中前几项是本次新收到的字节。Index是外面Loop提供的当前序号，从1开始；它不是已经收到的帧长度。
      | 
      | 1. 当前字节=Rx(Index)。Index≤Count时，本字节有效；否则只执行保持，不把数组尾部的旧值当作新字节。
      | 2. Index≥Count，或者Index=64，任一成立就输出“本批处理结束”。前者表示本批有效字节用完，后者防止超出64项。
      | 3. 尚未结束时输出下一序号Index+1；结束时输出65，让Loop退出。
      | 
      | 例如Count=3，依次处理数组第1、2、3项；到第3项就结束，不再把第4项作为新数据。Count=0时仍会有一次无效项处理，用于保持命令和处理通知，但不会往帧里加入字节。
      | 
      | 本步骤只负责遍历接收数组；它不判断AA55帧头，不校验，不保存命令。Byte和Active送第二步，Last送第五步，NextIndex反馈Loop。
  Step02_拼帧并记住未收完的数据 : Subsystem  Description=|
      | 第二步：识别帧头、拼满14字节，并记住半帧
      | 
      | 输入是一项字节及“本字节有效”标志。内部Collect按AA、55识别帧头，接着按顺序把后续字节放进14项候选缓存，收齐时给出Complete。
      | 
      | Buffer保存尚未验证的候选内容，Position保存下一项要放的位置。每个字节处理后，新的缓存与位置经过类型转换存回记忆，供下一个字节使用；本批结束时也不清掉，因此可跨接收批次续收。
      | 
      | 例：第一次只收到AA、55及其后6字节，第二次又收到剩余6字节，第二次会继续原位置，直到拼满14字节。无效项不会推进收帧。
      | 
      | 输出“候选帧”只是凑齐的内容，尚不能当命令使用；输出“本字节刚好收齐”是一次完成事件。两者送第三步校验，候选内容也送第四步等待是否接受。
      | 
      | 这里的延迟按循环处理的节奏保存记忆，不是在每个字节之间额外等待1 ms。更细的帧头重同步规则仍在Collect内部，原逻辑未改。
  Step03_检查完整性与双校验 : Subsystem  Description=|
      | 第三步：这一帧既要收齐，也要两种校验都通过
      | 
      | Verify只对已收齐的14字节候选帧作有效性检查。对第1～12字节重新计算：
      | 累加校验=这12字节之和 mod 256；
      | 异或校验=第1字节 XOR 第2字节 XOR … XOR 第12字节。
      | 分别与第13、第14字节比较，两项均匹配才通过。
      | 
      | 最终接受事件=“本字节刚好收齐” AND “Verify通过”。即使Verify保留着上一帧的通过状态，没有本次Complete也不会再次接受旧内容。
      | 
      | 例如数据未收满、累加校验不符、异或校验不符，任意一种都会使本次接受事件为假。为真时通知第四步更新命令，并通知第五步记住有新命令待报告。
      | 
      | 本处检查的是通信内容是否符合校验，不判断某条起动命令在当前发动机状态下是否允许执行；命令解释与模式判断在后面的CMMRead、ESM。
  Step04_只保存通过校验的命令 : Subsystem  Description=|
      | 第四步：只用有效帧更新命令，坏帧不能覆盖好命令
      | 
      | 将14字节候选帧后面补36个0，保持原工程50项命令接口：前14项是收到的帧，15～50项为兼容占位。
      | 
      | 本次接受事件为真：选择这组新命令，并存入Latest；
      | 本次接受事件为假：继续输出Latest记住的旧命令。
      | 
      | 例如上一条有效命令是A，本批又来了校验错误的B，输出仍为A；B不会因为已经凑满14字节就覆盖A。首次尚未接受命令时，沿用原有初始值。
      | 
      | 一个接收批次可能连续有多条有效帧，每接受一条就更新一次，批次结束后输出最后一条。这个50项数组是最近有效结果，不是每次通知就自动清空的队列。
      | 
      | 输出交外层Command。是否让控制任务在本拍使用它，由第五步的通知Flag另行表示。
  Step05_等到20毫秒再通知一次 : Subsystem  Description=|
      | 第五步：记住新命令，等20 ms更新时机再通知
      | 
      | Accepted表示本字节刚接受了有效帧，Fresh表示以前收到了有效帧但尚未报告。两者用OR合成NewSeen：只要其中一个为真，就说明有新命令等着通知。
      | 
      | 输出Flag=ControlTick AND NewSeen，再转成原接口数据类型。ControlTick由外层给出，表示当前到了20 ms更新时机；本步骤自己不计时，也不把秒数当输入。
      | 
      | 记忆更新：只有“本批处理结束 AND ControlTick”同时成立，才把待通知标志清零；其余时候继续保存NewSeen。这样循环尚未处理完时不会过早丢掉通知。
      | 
      | 例：第5 ms收到了有效帧，命令先被第四步保存，待通知状态保持；第20 ms更新许可到来时给出Flag，批次处理结束后清除。若这期间没有新帧，第40 ms不会再通知一次。
      | 
      | 同一更新间隔内收到多帧，通知表示“有更新”，第四步给出最近一条，不为每一帧单独排队。Flag是给控制任务的通知，不是向上位机发送的应答。
  Flag（20毫秒新命令通知）_106 : Outport
  Command（最近有效命令）_107 : Outport  Port=2
  wires:
  Step05_等到20毫秒再通知一次/1(新命令通知) -> Flag（20毫秒新命令通知）_106/1  "20毫秒新命令通知"
  Step04_只保存通过校验的命令/1(最近有效命令_50字节) -> Command（最近有效命令）_107/1  "最近有效命令_50项"
  Step01_取字节与循环控制/4(下一循环序号) -> Loop（逐项处理循环）_14/1  "下一序号或退出值65"
  ControlTick（20毫秒更新许可）_13/1 -> Step05_等到20毫秒再通知一次/3(20毫秒更新许可)  "20毫秒更新许可"
  Step01_取字节与循环控制/3(本批处理结束) -> Step05_等到20毫秒再通知一次/2(本批处理结束)  "本批最后一次循环"
  Step03_检查完整性与双校验/1(本字节接受新命令) -> Step04_只保存通过校验的命令/1(本字节接受新命令), Step05_等到20毫秒再通知一次/1(本字节接受新命令)  "本次接受有效帧"
  Step02_拼帧并记住未收完的数据/1(候选14字节帧) -> Step03_检查完整性与双校验/2(候选14字节帧), Step04_只保存通过校验的命令/2(候选14字节帧)  "候选14字节帧"
  Step02_拼帧并记住未收完的数据/2(本字节刚好收齐) -> Step03_检查完整性与双校验/1(本字节刚好收齐)  "刚好收齐一帧"
  Step01_取字节与循环控制/2(本字节有效) -> Step02_拼帧并记住未收完的数据/2(本字节有效)  "本项有效"
  Step01_取字节与循环控制/1(当前字节) -> Step02_拼帧并记住未收完的数据/1(当前字节)  "本项字节"
  Loop（逐项处理循环）_14/1 -> Step01_取字节与循环控制/3(当前循环序号)  "当前字节序号"
  Count（本次有效字节数）_12/1 -> Step01_取字节与循环控制/2(本批有效字节数)  "本批有效字节数"
  Rx（本次接收字节）_11/1 -> Step01_取字节与循环控制/1(接收缓冲_最多64字节)  "本批接收数组"

== system turbo_controller/BoardInput_输入换算与协议解析/In02_Motor（电机反馈解析）/Receive（逐字节组帧与保持有效结果）_235 ==
  note: 电机反馈接收流程：按1→2→3→4阅读
      |
      | 第一步只遍历本批有效字节，最多处理64项；第二步识别AA55、收齐9字节，并保存尚未收完的半帧；
      | 第三步确认本字节刚收齐且CRC通过；第四步换算数值并保存最近有效结果。
      |
      | Loop在一次调用内逐字节重复这些步骤，不是每一步各等1 ms。接收数组的Index每批重新遍历，收帧P
      | osition可以跨批保留，两者不是同一个位置。
      |
      | 有效帧第6、7字节合成整数，再除3向下取整得到电机反馈；没有有效新帧时保持旧值。
      |
      | 本次将原有处理块按职责封装，保留原协议、初始化、数据类型、校验和循环行为。各步骤内部可看输
      | 入、公式和例子。
  Rx（本次接收字节）_113 : Inport  OutDataTypeStr=uint8
  Count（本次有效字节数）_114 : Inport  Port=2  OutDataTypeStr=uint32
  Loop（逐项处理循环）_115 : ForIterator  IterationLimit=64  ExternalIncrement=on  IterationVariableDataType=uint32
  Step01_取字节与循环控制 : Subsystem  Description=|
      | 第一步：只处理本批收到的字节
      | 
      | 接收数组最多64项，Count是这次新收到的数量，Loop给出从1开始的Index。Byte=Rx(Index)，Active=(Index≤Count)。
      | 
      | 处理到Index≥Count或Index=64，就把下一循环序号设65，使Loop退出；否则下一序号=Index+1。Count=3只处理第1～3项；Count=0时仍走一次无效项保持路径，但不会把数组旧值加入帧。
      | 
      | 输出Byte和Active给组帧步骤，下一序号反馈Loop。这里不识别帧头，不作CRC，不把Index当作跨批收帧位置。
  Step02_拼帧并保存半帧 : Subsystem  Description=|
      | 第二步：跨多次接收保存半帧
      | 
      | 将本项字节、有效标志、上次候选缓存和上次收帧Position交给Collect。Collect识别AA55并逐项填满9字节，具体规则已在其内部再拆成五步。
      | 
      | 更新后的缓存和Position经原数据类型转换，送回两条记忆块；所以第一次只收到一半，下一批还能接着填，不必从头找AA。输出候选帧与“本字节刚收齐”，交第三步校验。
      | 
      | 候选缓存不等于已接受结果。即使旧缓存里已经有完整内容，没有本次收齐事件也不能再次接受它。这里的记忆按原循环节奏推进，没有增加一个额外的采样周期等待。
  Step03_收齐且校验通过才接受 : Subsystem  Description=|
      | 第三步：刚收齐且CRC通过，才接受新帧
      | 
      | Complete表示这一项字节刚把9字节补齐，先按原类型传给Verify触发校验。Verify对第6～7字节计算CRC16，分别与第8、9字节的高、低校验字节比较。
      | 
      | 最后Accepted=Complete AND Verify通过。这样未收齐的数据不会被采用，Verify上一帧保留的通过状态也不会在没有新Complete时重新接收旧帧。
      | 
      | CRC初值、表和覆盖范围保留原设置。校验失败只让本次Accepted为假；后面的保持步骤继续输出上一有效反馈。本处不作反馈比例换算，不直接生成驱动命令。
  Step04_换算反馈并保持有效结果 : Subsystem  Description=|
      | 第四步：把电机有效帧换算成反馈，并保持结果
      | 
      | 取候选帧第6字节为高字节、第7字节为低字节，先转成可运算类型，再计算：
      | 原始整数=第6字节×256+第7字节；
      | 候选反馈=floor(原始整数/3)。
      | 例如高1、低44合成300，除3后输出100。除3与向下取整均沿用原协议。
      | 
      | Accepted为真才更新输出和Motor记忆；为假则直接用旧值。坏帧或半帧不会覆盖上一有效反馈，同批多帧会按字节顺序逐次更新，最终保留最后一条。
      | 
      | 输出交外层测速来源选择。本步骤不发送电机命令，也不证明反馈没有超时；来源与超时判断仍在In05_Speed中完成。
  Speed（当前有效反馈）_234 : Outport
  wires:
  Count（本次有效字节数）_114/1 -> Step01_取字节与循环控制/2(输入2_本批有效字节数)  "本批有效字节数"
  Step02_拼帧并保存半帧/2(输出2_候选帧缓存) -> Step04_换算反馈并保持有效结果/1(输入1_候选帧缓存), Step03_收齐且校验通过才接受/2(输入2_候选帧缓存)  "候选帧缓存"
  Step01_取字节与循环控制/2(输出2_本项字节有效) -> Step02_拼帧并保存半帧/2(输入2_本项字节有效)  "本项字节有效"
  Rx（本次接收字节）_113/1 -> Step01_取字节与循环控制/3(输入3_本批接收数组)  "本批接收数组"
  Step01_取字节与循环控制/1(输出1_本项字节) -> Step02_拼帧并保存半帧/1(输入1_本项字节)  "本项字节"
  Step01_取字节与循环控制/3(输出3_下一循环序号) -> Loop（逐项处理循环）_115/1
  Step02_拼帧并保存半帧/1(输出1_本字节刚收齐) -> Step03_收齐且校验通过才接受/1(输入1_本字节刚收齐)  "本字节刚收齐"
  Loop（逐项处理循环）_115/1 -> Step01_取字节与循环控制/1(输入1_本批循环序号)  "本批循环序号"
  Step03_收齐且校验通过才接受/1(输出1_本字节接受有效帧) -> Step04_换算反馈并保持有效结果/2(输入2_本字节接受有效帧)  "本字节接受有效帧"
  Step04_换算反馈并保持有效结果/1(输出1_最近有效反馈) -> Speed（当前有效反馈）_234/1

== system turbo_controller/BoardInput_输入换算与协议解析/In03_Pump（油泵回包预留校验）/Receive（逐字节组帧与保持有效结果）_353 ==
  note: 预留油泵校验接收流程：按1→2→3→4阅读
      |
      | 第一步只遍历本批有效字节，最多处理64项；第二步识别AA55、收齐22字节，并保存尚未收完的半帧；
      | 第三步确认本字节刚收齐且CRC通过；第四步统计这一批是否出现过有效帧。
      |
      | Loop在一次调用内逐字节重复这些步骤，不是每一步各等1 ms。接收数组的Index每批重新遍历，收帧P
      | osition可以跨批保留，两者不是同一个位置。
      |
      | 本分支输出本批是否出现有效帧，不生成实际平滑泵速。实际泵速来自BoardOutput/Out01_Pump的接收
      | 路径。
      |
      | 本次将原有处理块按职责封装，保留原协议、初始化、数据类型、校验和循环行为。各步骤内部可看输
      | 入、公式和例子。
  Rx（本次接收字节）_239 : Inport  OutDataTypeStr=uint8
  Count（本次有效字节数）_240 : Inport  Port=2  OutDataTypeStr=uint32
  Loop（逐项处理循环）_241 : ForIterator  IterationLimit=64  ExternalIncrement=on  IterationVariableDataType=uint32
  Step01_取字节与循环控制 : Subsystem  Description=|
      | 第一步：只处理本批收到的字节
      | 
      | 接收数组最多64项，Count是这次新收到的数量，Loop给出从1开始的Index。Byte=Rx(Index)，Active=(Index≤Count)。
      | 
      | 处理到Index≥Count或Index=64，就把下一循环序号设65，使Loop退出；否则下一序号=Index+1。Count=3只处理第1～3项；Count=0时仍走一次无效项保持路径，但不会把数组旧值加入帧。
      | 
      | 输出Byte和Active给组帧步骤，下一序号反馈Loop。这里不识别帧头，不作CRC，不把Index当作跨批收帧位置。
  Step02_拼帧并保存半帧 : Subsystem  Description=|
      | 第二步：跨多次接收保存半帧
      | 
      | 将本项字节、有效标志、上次候选缓存和上次收帧Position交给Collect。Collect识别AA55并逐项填满22字节，具体规则已在其内部再拆成五步。
      | 
      | 更新后的缓存和Position经原数据类型转换，送回两条记忆块；所以第一次只收到一半，下一批还能接着填，不必从头找AA。输出候选帧与“本字节刚收齐”，交第三步校验。
      | 
      | 候选缓存不等于已接受结果。即使旧缓存里已经有完整内容，没有本次收齐事件也不能再次接受它。这里的记忆按原循环节奏推进，没有增加一个额外的采样周期等待。
  Step03_收齐且校验通过才接受 : Subsystem  Description=|
      | 第三步：刚收齐且CRC通过，才接受新帧
      | 
      | Complete表示这一项字节刚把22字节补齐，先按原类型传给Verify触发校验。Verify对第6～20字节计算CRC16，分别与第21、22字节的高、低校验字节比较。
      | 
      | 最后Accepted=Complete AND Verify通过。这样未收齐的数据不会被采用，Verify上一帧保留的通过状态也不会在没有新Complete时重新接收旧帧。
      | 
      | CRC初值、表和覆盖范围保留原设置。校验失败只让本次Accepted为假；后面的批次统计继续看这一批有没有其他有效帧。本处不作反馈比例换算，不直接生成驱动命令。
  Step04_统计本批是否有有效帧 : Subsystem  Description=|
      | 第四步：统计本批有没有接受过有效帧
      | 
      | 根据Loop的Index判断是不是本批第一项。第一项先把累计结果视为false，后续项继续采用Seen记忆；再把这个累计结果与本项Accepted作OR。
      | 
      | 只要这一批某项收齐并校验通过，后面即使是普通字节或无效帧，批次结果仍保持true；下一批会在第一项重新统计。它不是跨所有批次永久锁存的有效标志。
      | 
      | 例如本批先坏帧、后好帧，最后输出true；整批没有好帧则false。此分支只输出校验统计，不计算泵速，也没有0.875/0.125滤波，不能与BoardOutput内的实际泵反馈路径混淆。
  Valid（原预留校验结果）_352 : Outport
  wires:
  Count（本次有效字节数）_240/1 -> Step01_取字节与循环控制/2(输入2_本批有效字节数)  "本批有效字节数"
  Step02_拼帧并保存半帧/2(输出2_候选帧缓存) -> Step03_收齐且校验通过才接受/2(输入2_候选帧缓存)  "候选帧缓存"
  Step01_取字节与循环控制/2(输出2_本项字节有效) -> Step02_拼帧并保存半帧/2(输入2_本项字节有效)  "本项字节有效"
  Rx（本次接收字节）_239/1 -> Step01_取字节与循环控制/3(输入3_本批接收数组)  "本批接收数组"
  Step01_取字节与循环控制/1(输出1_本项字节) -> Step02_拼帧并保存半帧/1(输入1_本项字节)  "本项字节"
  Step02_拼帧并保存半帧/1(输出1_本字节刚收齐) -> Step03_收齐且校验通过才接受/1(输入1_本字节刚收齐)  "本字节刚收齐"
  Loop（逐项处理循环）_241/1 -> Step04_统计本批是否有有效帧/2(输入2_本批循环序号), Step01_取字节与循环控制/1(输入1_本批循环序号)  "本批循环序号"
  Step01_取字节与循环控制/3(输出3_下一循环序号) -> Loop（逐项处理循环）_241/1
  Step03_收齐且校验通过才接受/1(输出1_本字节接受有效帧) -> Step04_统计本批是否有有效帧/1(输入1_本字节接受有效帧)  "本字节接受有效帧"
  Step04_统计本批是否有有效帧/1(输出1_本批出现过有效帧) -> Valid（原预留校验结果）_352/1

== system turbo_controller/BoardInput_输入换算与协议解析/In04_Capture（捕获间隔缓存）/Step01_逐项取出本批有效捕获 ==
  note: 第一步：按顺序取出本批捕获，不处理数组尾部旧值
      |
      | 外层Loop给出从1开始的序号i。本项捕获=Capture(i)，本项有效=(i≤本批Count)。
      |
      | 如果i已达到本批Count，或i=16，就把下一循环序号设17，结束循环；否则下一序号=i+1。因此输入数
      | 组虽然有16项，Count=3时只会把前3项当新捕获。Count=0时保留一次无效项处理，状态由后面保持，
      | 不写入新间隔。
      |
      | 例：一批有[1000,2000,3000]三项，依次交给更新步骤处理；它们是在本次调用内顺序处理，不是分三
      | 毫秒执行。
      |
      | 输出分别为本项捕获、有效许可和下一循环序号。i是本批数组位置，不是十项环形缓存的写入位置。
  输入1_本批当前处理序号 : Inport
  输入2_本批有效捕获个数 : Inport  Port=2
  输入3_本批最多16项捕获数组 : Inport  Port=3
  Active（本项在有效范围内）_359 : RelationalOperator  Operator=<=  OutDataTypeStr=boolean  RndMeth=Simplest  InputSameDT=off
  Add（加减运算）_366 : Sum  SaturateOnIntegerOverflow=on  OutDataTypeStr=Inherit: Same as first input
  AtLimit（达到处理上限）_362 : RelationalOperator  Operator===  OutDataTypeStr=boolean  RndMeth=Simplest  InputSameDT=off
  Constant（常量）_361 : Constant  Value=16  OutDataTypeStr=uint32
  Constant（常量）_364 : Constant  Value=17  OutDataTypeStr=uint32
  Constant（常量）_365 : Constant  OutDataTypeStr=uint32
  Last（本周期最后一项）_363 : Logic  Operator=OR  IconShape=distinctive  AllPortsSameDT=off  OutDataTypeStr=boolean
  NextIndex（处理下一项或结束）_367 : Switch  Criteria=u2 ~= 0  SaturateOnIntegerOverflow=off  InputSameDT=off
  ReceivedAll（已处理所有有效项）_360 : RelationalOperator  OutDataTypeStr=boolean  RndMeth=Simplest  InputSameDT=off
  Select（按索引取元素）_373 : Selector  InputPortWidth=16  IndexOptions=Index vector (port)  Indices=1  OutputSizes=1
  输出1_下一序号或退出值17 : Outport
  输出2_本项捕获读数 : Outport  Port=2
  输出3_本项捕获有效 : Outport  Port=3
  wires:
  Active（本项在有效范围内）_359/1 -> 输出3_本项捕获有效/1
  Select（按索引取元素）_373/1 -> 输出2_本项捕获读数/1
  NextIndex（处理下一项或结束）_367/1 -> 输出1_下一序号或退出值17/1
  输入3_本批最多16项捕获数组/1 -> Select（按索引取元素）_373/1
  Add（加减运算）_366/1 -> NextIndex（处理下一项或结束）_367/3
  Last（本周期最后一项）_363/1 -> NextIndex（处理下一项或结束）_367/2
  Constant（常量）_364/1 -> NextIndex（处理下一项或结束）_367/1
  AtLimit（达到处理上限）_362/1 -> Last（本周期最后一项）_363/2
  ReceivedAll（已处理所有有效项）_360/1 -> Last（本周期最后一项）_363/1
  Constant（常量）_361/1 -> AtLimit（达到处理上限）_362/2
  Constant（常量）_365/1 -> Add（加减运算）_366/2
  输入2_本批有效捕获个数/1 -> ReceivedAll（已处理所有有效项）_360/2, Active（本项在有效范围内）_359/2
  输入1_本批当前处理序号/1 -> ReceivedAll（已处理所有有效项）_360/1, Select（按索引取元素）_373/2, Active（本项在有效范围内）_359/1, AtLimit（达到处理上限）_362/1, Add（加减运算）_366/1

== system turbo_controller/BoardInput_输入换算与协议解析/In04_Capture（捕获间隔缓存）/Step02_保存捕获与缓存历史状态 ==
  note: 第二步：保留下一项计算还要用到的五种历史状态
      |
      | 这里的五条记忆各有用途：
      | Previous：上一项有效捕获读数，用来求下一次差分，初值0；
      | Ring：最近十个已接受间隔，初值为十个0；
      | Index：下一次覆盖缓存的哪一项，初值1；
      | Count：已保存多少个有效间隔，初值0，最多10；
      | LastTime：最近接受正间隔的处理时刻，初值-1秒。
      |
      | 每次把Step03给出的新状态按原类型保存：Previous为uint32，Index和Count为uint8，Ring和LastTim
      | e为single；下一次循环/调用再提供给Step03。
      |
      | 不要把Previous、Ring和LastTime混为一份数据。读数用于差分，间隔用于测速，时间用于判断新鲜程
      | 度。没有有效捕获时，上游选择器会把旧状态送回来，记忆继续保持。
  输入1_更新后的十项间隔 : Inport
  输入2_最近有效间隔处理时刻 : Inport  Port=2
  输入3_下一差分基准 : Inport  Port=3
  输入4_下一环形写入位置 : Inport  Port=4
  输入5_更新后的有效间隔数 : Inport  Port=5
  Count（已保存的有效间隔数）_371 : UnitDelay  InitialCondition=uint8(0)  SampleTime=-1  HasFrameUpgradeWarning=on
  Index（环形缓存写入位置）_370 : UnitDelay  InitialCondition=uint8(1)  SampleTime=-1  HasFrameUpgradeWarning=on
  LastTime（最近有效脉冲秒数）_372 : UnitDelay  InitialCondition=single(-1)  SampleTime=-1  HasFrameUpgradeWarning=on
  Previous（上次捕获计数）_368 : UnitDelay  InitialCondition=uint32(0)  SampleTime=-1  HasFrameUpgradeWarning=on
  Ring（跨周期十项间隔缓存）_369 : UnitDelay  InitialCondition=single(zeros(10,1))  SampleTime=-1  HasFrameUpgradeWarning=on
  Store_single（按单精度数保存状态）_536830 : DataTypeConversion  Description=为反馈回路显式指定原程序的状态类型，保持原状态更新节拍。  OutDataTypeStr=single  RndMeth=Round
  Store_single（按单精度数保存状态）_536833 : DataTypeConversion  Description=为反馈回路显式指定原程序的状态类型，保持原状态更新节拍。  OutDataTypeStr=single  RndMeth=Round
  Store_uint32（按三十二位无符号数保存状态）_536829 : DataTypeConversion  Description=为反馈回路显式指定原程序的状态类型，保持原状态更新节拍。  OutDataTypeStr=uint32  RndMeth=Round
  Store_uint8（按八位无符号数保存状态）_536831 : DataTypeConversion  Description=为反馈回路显式指定原程序的状态类型，保持原状态更新节拍。  OutDataTypeStr=uint8  RndMeth=Round
  Store_uint8（按八位无符号数保存状态）_536832 : DataTypeConversion  Description=为反馈回路显式指定原程序的状态类型，保持原状态更新节拍。  OutDataTypeStr=uint8  RndMeth=Round
  输出1_上一捕获读数 : Outport
  输出2_旧十项间隔缓存 : Outport  Port=2
  输出3_当前环形写入位置 : Outport  Port=3
  输出4_累计有效间隔数 : Outport  Port=4
  输出5_上次有效间隔时刻 : Outport  Port=5
  wires:
  LastTime（最近有效脉冲秒数）_372/1 -> 输出5_上次有效间隔时刻/1
  Count（已保存的有效间隔数）_371/1 -> 输出4_累计有效间隔数/1
  Index（环形缓存写入位置）_370/1 -> 输出3_当前环形写入位置/1
  Ring（跨周期十项间隔缓存）_369/1 -> 输出2_旧十项间隔缓存/1
  Previous（上次捕获计数）_368/1 -> 输出1_上一捕获读数/1
  输入5_更新后的有效间隔数/1 -> Store_uint8（按八位无符号数保存状态）_536832/1
  输入4_下一环形写入位置/1 -> Store_uint8（按八位无符号数保存状态）_536831/1
  输入3_下一差分基准/1 -> Store_uint32（按三十二位无符号数保存状态）_536829/1
  输入2_最近有效间隔处理时刻/1 -> Store_single（按单精度数保存状态）_536833/1
  输入1_更新后的十项间隔/1 -> Store_single（按单精度数保存状态）_536830/1
  Store_single（按单精度数保存状态）_536830/1 -> Ring（跨周期十项间隔缓存）_369/1
  Store_uint32（按三十二位无符号数保存状态）_536829/1 -> Previous（上次捕获计数）_368/1
  Store_single（按单精度数保存状态）_536833/1 -> LastTime（最近有效脉冲秒数）_372/1
  Store_uint8（按八位无符号数保存状态）_536831/1 -> Index（环形缓存写入位置）_370/1
  Store_uint8（按八位无符号数保存状态）_536832/1 -> Count（已保存的有效间隔数）_371/1
